simulink model "HybridShip_ModelD_DCBus"  (R2026a)
settings: Solver=ode3  StopTime=7200  FixedStep=0.01
undefined symbols (not defined in the file): AI_Pred_Source, AI_TPeak_Source, ASSUMED_AI_DataValid, ASSUMED_Bat_ChargeLimit, ASSUMED_Bat_DischargeLimit, ASSUMED_Bat_Eff_Charge, ASSUMED_Bat_Eff_Discharge, ASSUMED_BSFC_Breakpoints, ASSUMED_BSFC_Table, ASSUMED_C_bus, ASSUMED_Drive_TimeConstant, ASSUMED_EMS_FF_Gain, ASSUMED_EMS_FF_Max_kW, ASSUMED_EMS_Manual_Pgen_kW, ASSUMED_EMS_SOC_Gain, ASSUMED_EMS_SOC_Ref, ASSUMED_eta_dcdc, ASSUMED_eta_rect, ASSUMED_Gen_MinStablePower, ASSUMED_Gen_TimeConstant, ASSUMED_K_droop, ASSUMED_Pred_Bound_kW, ASSUMED_SOC_ChgDerate_Start, ASSUMED_SOC_DisDerate_Start, ASSUMED_SOC_max, ASSUMED_SOC_min, ASSUMED_SpeedPI_Ki, ASSUMED_SpeedPI_Kp, ASSUMED_TFF_SOC_AdvancePct, ASSUMED_TFF_SOC_Thresh, ASSUMED_TFF_TauMargin, ASSUMED_V_floor, Bat_Cap_kWh, Bat_SOC_init, BSFC_Breakpoints_kW, BSFC_Table_gkWh, CCS_Vdc_Steady_Band, CCS_Vdc_Transient_Band, ECMS_dt_ctrl_s, ECMS_Grid_dP_kW, ECMS_Idle_Fuel_kgph, ECMS_K_S, ECMS_K_soc, ECMS_Lambda, ECMS_Lambda_Floor, ECMS_NN_b1, ECMS_NN_b2, ECMS_NN_b3, ECMS_NN_Ebar_H_kWh, ECMS_NN_Escale_kWh, ECMS_NN_W1, ECMS_NN_W2, ECMS_NN_W3, ECMS_NN_WeightsOK, ECMS_NN_XMean, ECMS_NN_XStd, ECMS_NN_YMean, ECMS_NN_YStd, ECMS_SOC_Charge_Min, ECMS_SOC_Discharge_Max ... (+43)
libraries: simulink x3
(part 3 of 3)

== matlab function HybridShip_ModelD_DCBus/14_Battery_Converter/bat_limits ==
  data: SOC input; dis output; chg output; ASSUMED_SOC_min parameter; ASSUMED_SOC_max parameter; ASSUMED_SOC_DisDerate_Start parameter; ASSUMED_SOC_ChgDerate_Start parameter; ASSUMED_Bat_DischargeLimit parameter; ASSUMED_Bat_ChargeLimit parameter
function [dis, chg] = bat_limits(SOC, ASSUMED_SOC_min, ASSUMED_SOC_max, ASSUMED_SOC_DisDerate_Start, ASSUMED_SOC_ChgDerate_Start, ASSUMED_Bat_DischargeLimit, ASSUMED_Bat_ChargeLimit)
% 电池充放电可用功率（SOC 降额）
if SOC <= ASSUMED_SOC_min
    dis = 0;
elseif SOC >= ASSUMED_SOC_DisDerate_Start
    dis = ASSUMED_Bat_DischargeLimit;
else
    dis = ASSUMED_Bat_DischargeLimit * (SOC - ASSUMED_SOC_min) / ...
        (ASSUMED_SOC_DisDerate_Start - ASSUMED_SOC_min);
end
if SOC >= ASSUMED_SOC_max
    chg = 0;
elseif SOC <= ASSUMED_SOC_ChgDerate_Start
    chg = ASSUMED_Bat_ChargeLimit;
else
    chg = ASSUMED_Bat_ChargeLimit * (ASSUMED_SOC_max - SOC) / ...
        (ASSUMED_SOC_max - ASSUMED_SOC_ChgDerate_Start);
end
end

== matlab function HybridShip_ModelD_DCBus/14_Battery_Converter/soc_rate ==
  data: P_bus input; r output; Bat_Cap_kWh parameter; ASSUMED_Bat_Eff_Discharge parameter; ASSUMED_Bat_Eff_Charge parameter; ASSUMED_eta_dcdc parameter
function r = soc_rate(P_bus, Bat_Cap_kWh, ASSUMED_Bat_Eff_Discharge, ASSUMED_Bat_Eff_Charge, ASSUMED_eta_dcdc)
% SOC 变化率：P_bus 为母线侧功率；先折算到电池端（含 DC/DC 效率）
E = Bat_Cap_kWh * 3600;
if P_bus > 0
    P_term = P_bus / ASSUMED_eta_dcdc;
    r = -(P_term / ASSUMED_Bat_Eff_Discharge) / E;
else
    P_term = P_bus * ASSUMED_eta_dcdc;
    r = -P_term * ASSUMED_Bat_Eff_Charge / E;
end
end

== matlab function HybridShip_ModelD_DCBus/08_Undervolt_Derate/derate_fn ==
  data: V input; f output; CCS_Vdc_Steady_Band parameter; CCS_Vdc_Transient_Band parameter
function f = derate_fn(V, CCS_Vdc_Steady_Band, CCS_Vdc_Transient_Band)
% 欠压降额系数：CCS 稳态下限以上 f=1，线性降至瞬态下限 f=0
v_lo = CCS_Vdc_Transient_Band(1);
v_hi = CCS_Vdc_Steady_Band(1);
f = min(max((V - v_lo) / (v_hi - v_lo), 0), 1);
end

== matlab function HybridShip_ModelD_DCBus/13_DC_Bus/dVdt ==
  data: P_res_kW input; dv output; V input; ASSUMED_C_bus parameter; ASSUMED_V_floor parameter
function dv = dVdt(P_res_kW, V, ASSUMED_C_bus, ASSUMED_V_floor)
% 母线电压动态：C*V*dV/dt = P_res（kW -> W 换算，V_floor 除法保护）
dv = P_res_kW * 1000 / (ASSUMED_C_bus * max(V, ASSUMED_V_floor));
end

== matlab function HybridShip_ModelD_DCBus/15_Bus_Voltage_Monitor/ccs_check ==
  data: V input; al_s output; al_t output; CCS_Vdc_Steady_Band parameter; CCS_Vdc_Transient_Band parameter
function [al_s, al_t] = ccs_check(V, CCS_Vdc_Steady_Band, CCS_Vdc_Transient_Band)
% CCS 2026 电能质量判定：稳态带 -10%/+6%，瞬态带 -20%/+7%
al_s = double(V < CCS_Vdc_Steady_Band(1) || V > CCS_Vdc_Steady_Band(2));
al_t = double(V < CCS_Vdc_Transient_Band(1) || V > CCS_Vdc_Transient_Band(2));
end

== matlab function HybridShip_ModelD_DCBus/01_Scenario_Manager/current_profile ==
  data: x input; vc output; t input; mode input; kx input; kv input; v_def input; tt input; tv input
function vc = current_profile(x, t, mode, kx, kv, v_def, tt, tv)
% 水流速度剖面：mode=0 按里程节点分段线性（既有；负=逆水，正=顺水，节点 -1 结束）
% mode=1 按时间节点分段恒定（S20：仅段 9 逆水 -1 m/s，其余 0）
if mode > 0.5
    vc = v_def;
    if tt(1) < 0
        return;
    end
    if t <= tt(1)
        vc = tv(1);
        return;
    end
    for k = 1:numel(tt)-1
        if t < tt(k+1)
            vc = tv(k);
            return;
        end
    end
    vc = tv(end);
    return;
end
vc = v_def;
if kx(1) < 0
    return;
end
if x <= kx(1)
    vc = kv(1);
    return;
end
for k = 1:3
    if kx(k+1) < 0
        vc = kv(k);
        return;
    end
    if x <= kx(k+1)
        w = (x - kx(k)) / max(kx(k+1) - kx(k), 1e-6);
        vc = kv(k) + w * (kv(k+1) - kv(k));
        return;
    end
end
vc = kv(4);
end

== matlab function HybridShip_ModelD_DCBus/01_Scenario_Manager/v_cmd_profile ==
  data: x input; v output; t input; mode input; kx input; kv input; v_def input; tt input; tv input
function v = v_cmd_profile(x, t, mode, kx, kv, v_def, tt, tv)
% 目标航速剖面：mode=0 距离节点分段线性（既有语义）；mode=1 时间节点分段恒定（S20，design §2.1）
% 时间模式过渡由下游 Rate Limiter 按 SCN.accel/decel_ramp_mps2 平滑（以限幅器为准）
if mode > 0.5
    v = v_def;
    if tt(1) < 0
        return;
    end
    if t <= tt(1)
        v = tv(1);
        return;
    end
    for k = 1:numel(tt)-1
        if t < tt(k+1)
            v = tv(k);
            return;
        end
    end
    v = tv(end);
    return;
end
v = v_def;
if kx(1) < 0
    return;
end
if x <= kx(1)
    v = kv(1);
    return;
end
for k = 1:5
    if kx(k+1) < 0
        v = kv(k);
        return;
    end
    if x <= kx(k+1)
        w = (x - kx(k)) / max(kx(k+1) - kx(k), 1e-6);
        v = kv(k) + w * (kv(k+1) - kv(k));
        return;
    end
end
v = kv(6);
end

== matlab function HybridShip_ModelD_DCBus/01_Scenario_Manager/resist_profile ==
  data: x input; m output; profile input; pos input; amp input; rampT input; bands input; v_target input
function m = resist_profile(x, profile, pos, amp, rampT, bands, v_target)
% 阻力倍率剖面（距离触发，x 平滑过渡；无状态，适合连续采样）
% 过渡带宽度 = v_target * rampT（约 10~20 s 对应距离）；bands: 4x3 [起点 终点 幅值]，起点<0 结束
dx = v_target * max(rampT, 1e-6);
r = min(max((x - pos) / max(dx, 1e-6), 0), 1);
switch profile
    case 0
        m = 1;
    case 1
        m = 1 + amp * r;
    case 2
        m = 1 + amp * r;
    case 3
        if x >= pos, m = 1 + amp; else, m = 1; end
    case 4
        m = 1;
        for k = 1:4
            xs = bands(k, 1);
            if xs < 0
                break;
            end
            xe = bands(k, 2);
            a = bands(k, 3);
            r_up = min(max((x - xs) / max(dx, 1e-6), 0), 1);
            r_dn = min(max((x - xe) / max(dx, 1e-6), 0), 1);
            m = m + a * (r_up - r_dn);
        end
    otherwise
        m = 1;
end
m = max(m, 0.05);
end

== matlab function HybridShip_ModelD_DCBus/03_Propulsion_Plant/Propeller_Hydrodynamics ==
  data: n_prop_rpm input; F_prop_eff output; V_ship_mps input; V_current_mps input; Q_prop output; P_hydro_kW output; V_A output; wake_fraction parameter; K_Fw parameter; K_Fv parameter; K_Qw parameter; K_Qv parameter
function [F_prop_eff, Q_prop, P_hydro_kW, V_A] = PropellerHydroSimple(...
    n_prop_rpm, V_ship_mps, V_current_mps, wake_fraction, K_Fw, K_Fv, K_Qw, K_Qv)
% 简化螺旋桨水动力模型（复用原模型，未修改）
omega = n_prop_rpm * pi / 30;
V_rel = V_ship_mps - V_current_mps;
V_A = (1 - wake_fraction) * V_rel;
F_prop_eff = K_Fw * omega * abs(omega) - K_Fv * V_A * abs(V_A);
Q_prop = K_Qw * omega * abs(omega) - K_Qv * V_A * abs(V_A);
P_hydro_kW = Q_prop * omega / 1000;
end

== matlab function HybridShip_ModelD_DCBus/03_Propulsion_Plant/Ship_Hull_Dynamics ==
  data: V_ship input; dVdt output; F_prop_eff input; V_current input; F_env input; resistance_multiplier input; R_hull output; Hull_K_R parameter; Ship_Mass parameter
function [dVdt, R_hull] = HullLongitudinalDynamics(...
    V_ship, F_prop_eff, V_current, F_env, resistance_multiplier, Hull_K_R, Ship_Mass)
% 船体纵向动力学（原模型基础上增加阻力倍率输入）
V_rel = V_ship - V_current;
R_hull = resistance_multiplier * Hull_K_R * V_rel * abs(V_rel);
dVdt = (F_prop_eff - R_hull + F_env) / Ship_Mass;
end
